simulink model "manometer"  (R2025b)
settings: Solver=VariableStepAuto  StartTime=0.0  StopTime=3600  RelTol=1e-5  AbsTol=1e-7
libraries: fl_lib x17, customization_lib x5, nesl_utility x5
settings Model: Creator=degoede  LastModifiedBy=degoede
settings SolverCC: AutoScaleAbsTol=off
settings SimscapeCC: SimscapeLogType=all  SimscapeLogSimulationStatistics=on  SimscapeLogOpenViewer=on  SimscapeLogLimitData=off

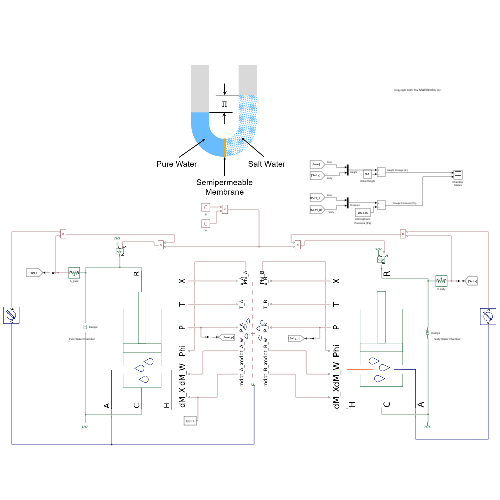
[thumbnail: Simulink's stored preview of the top-level diagram]
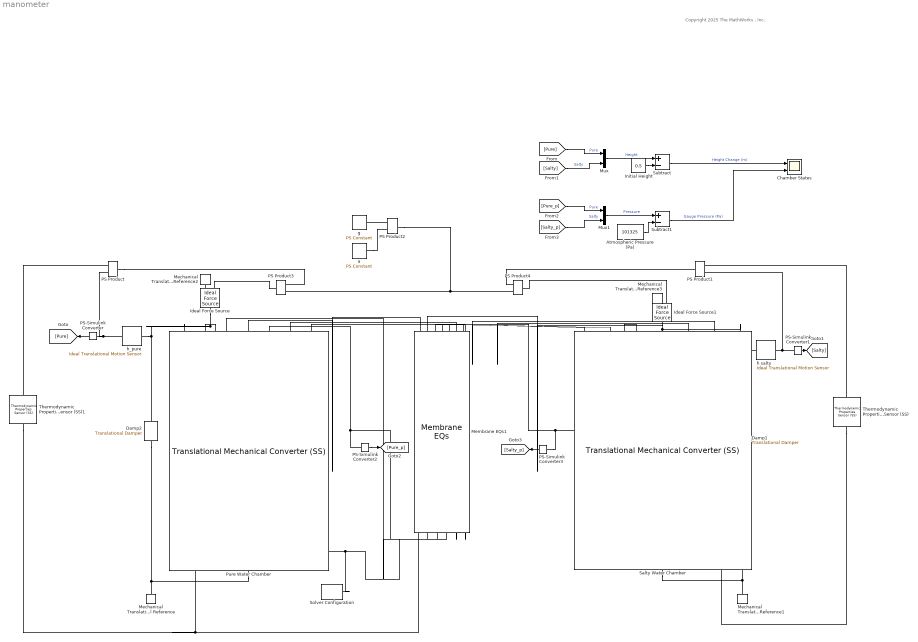
== system manometer ==
  note: Copyright 2025 The MathWorks , Inc.
  Atmospheric Pressure (Pa) : Constant  Value=101325
  Chamber States : Scope  NumInputPorts=2
      settings: Title=Gauge Pressure (Pa)  ActiveDisplayYMinimum=2584.7701229857284  ActiveDisplayYMaximum=6665.5615631627643
  Damp1 : fl_lib/Mechanical/Translational Elements/Translational Damper  D=0.001 N*s/m  v_specify=off  v_priority=None  v=0 m/s  v_nominal_specify=off  v_nominal_value=1  v_nominal_unit=m/s  f_specify=off  f_priority=None  f=0 N  f_nominal_specify=off  f_nominal_value=1  f_nominal_unit=N
  Damp2 : fl_lib/Mechanical/Translational Elements/Translational Damper  D=0.001 N*s/m  v_specify=off  v_priority=None  v=0 m/s  v_nominal_specify=off  v_nominal_value=1  v_nominal_unit=m/s  f_specify=off  f_priority=None  f=0 N  f_nominal_specify=off  f_nominal_value=1  f_nominal_unit=N
  Ideal Force Source : fl_lib/Mechanical/Mechanical Sources/Ideal Force Source
  Ideal Force Source1 : fl_lib/Mechanical/Mechanical Sources/Ideal Force Source
  Initial Height : Constant  Value=0.5
  Mechanical Translational Reference{,1..3} (4 alike) : fl_lib/Mechanical/Translational Elements/Mechanical Translational Reference
  Membrane EQs1 : customization_lib/membranes/Membrane EQs  A_w=2.57e-6 m^3/(N*s)  B_s=2.30e-8 m/s  A_m=1 cm^2
      settings: SourceProductName=Customization  InternalSimscapePortConfiguration="{\"Bottom\":[{\"id\":\"mdot_B_x\",\"label\":\"mdot_B_x\",\"type\":\"output\"},{\"id\":\"mdot_B_w\",\"label\":\"mdot_B_w\",\"type\":\"output\"},{\"id\":\"P_B\",\"label\":\"P_B\",\"type\":\"input\"},{\"id\":\"T_B\",\"label\":\"T_B\",\"type\":\"input\"},{\"id\":\"x_B\",\"label\":\"x_B\",\"type\":\"input\"}],\"Left\":[{\"id\":\"F\",\"label\":\"F\",\"type\":\"customization.solution.solution\"}],\"Right\":[{\"id\":\"Phi_A\",\"label\":\"Phi_A\",\"type\":\"output\"},{\"id\":\"Phi_B\",\"label\":\"Phi_B\",\"type\":\"output\"}],\"Top\":[{\"id\":\"mdot_A_x\",\"label\":\"mdot_A_x\",\"type\":\"output\"},{\"id\":\"mdot_A_w\",\"label\":\"mdot_A_w\",\"type\":\"output\"},{\"id\":\"P_A\",\"label\":\"P_A\",\"type\":\"input\"},{\"id\":\"T_A\",\"label\":\"T_A\",\"type\":\"input\"},{\"id\":\"x_A\",\"label\":\"x_A\",\"type\":\"input\"}]}"
  Mux : Mux  Inputs=2
  Mux1 : Mux  Inputs=2
  PS Product{,1..4} (5 alike) : fl_lib/Physical Signals/Functions/PS Product
  PS-Simulink Converter : nesl_utility/PS-Simulink Converter  PhysicalDomain=network_engine_domain  SubClassName=ps_output  LeftPortType=input  RightPortType=output  PseudoPeriodic=off  Frequencies=[]  VectorFormat=inherit  Unit=m  AffineConversion=off
  PS-Simulink Converter1 : nesl_utility/PS-Simulink Converter  PhysicalDomain=network_engine_domain  SubClassName=ps_output  LeftPortType=input  RightPortType=output  PseudoPeriodic=off  Frequencies=[]  VectorFormat=inherit  Unit=m  AffineConversion=off
  PS-Simulink Converter2 : nesl_utility/PS-Simulink Converter  PhysicalDomain=network_engine_domain  SubClassName=ps_output  LeftPortType=input  RightPortType=output  PseudoPeriodic=off  Frequencies=[]  VectorFormat=inherit  Unit=Pa  AffineConversion=off
  PS-Simulink Converter3 : nesl_utility/PS-Simulink Converter  PhysicalDomain=network_engine_domain  SubClassName=ps_output  LeftPortType=input  RightPortType=output  PseudoPeriodic=off  Frequencies=[]  VectorFormat=inherit  Unit=Pa  AffineConversion=off
  Pure Water Chamber : customization_lib/solution/elements/Translational Mechanical Converter (SS)  mech_orientation=foundation.enum.MechOrientationTranslational.Positive  length_init=0.5 m  interface_area=1 cm^2  dead_volume=1e-07 m^3  area_A=1 cm^2  pressure_spec=foundation.enum.pressure_spec.atmospheric  environment_pressure=0.101325 MPa  m_measure=false  p_measure=true  t_measure=true  x_measure=true  p_I_specify=on  p_I_priority=High  p_I=998.2*9.81*0.5/1e6 + 0.101325 MPa  p_I_nominal_specify=off  p_I_nominal_value=1  p_I_nominal_unit=MPa  T_I_specify=off  T_I_priority=High  T_I=293.15 K  T_I_nominal_specify=off  T_I_nominal_value=1  T_I_nominal_unit=K  x_I_specify=on  x_I_priority=High  x_I=0 kg/m^3  x_I_nominal_specify=off  x_I_nominal_value=1  x_I_nominal_unit=kg/m^3
      settings: SourceProductName=Customization  InternalSimscapePortConfiguration="{\"Bottom\":[{\"id\":\"dM_X\",\"label\":\"dM_X\",\"type\":\"input\"},{\"id\":\"dM_W\",\"label\":\"dM_W\",\"type\":\"input\"},{\"id\":\"Phi\",\"label\":\"Phi\",\"type\":\"input\"},{\"id\":\"P\",\"label\":\"P\",\"type\":\"output\"},{\"id\":\"T\",\"label\":\"T\",\"type\":\"output\"},{\"id\":\"X\",\"label\":\"X\",\"type\":\"output\"}],\"Left\":[{\"id\":\"A\",\"label\":\"A\",\"type\":\"customization.solution.solution\"},{\"id\":\"C\",\"label\":\"C\",\"type\":\"foundation.mechanical.translational.translational\"},{\"id\":\"H\",\"label\":\"H\",\"type\":\"foundation.thermal.thermal\"}],\"Right\":[{\"id\":\"R\",\"label\":\"R\",\"type\":\"foundation.mechanical.translational.translational\"}],\"Top\":[]}"
  Salty Water Chamber : customization_lib/solution/elements/Translational Mechanical Converter (SS)  mech_orientation=foundation.enum.MechOrientationTranslational.Positive  length_init=0.5 m  interface_area=1 cm^2  dead_volume=1e-07 m^3  area_A=1 cm^2  pressure_spec=foundation.enum.pressure_spec.atmospheric  environment_pressure=0.101325 MPa  m_measure=false  p_measure=true  t_measure=true  x_measure=true  p_I_specify=on  p_I_priority=High  p_I=998.25*9.81*0.5/1e6 + 0.101325 MPa  p_I_nominal_specify=off  p_I_nominal_value=1  p_I_nominal_unit=MPa  T_I_specify=off  T_I_priority=High  T_I=293.15 K  T_I_nominal_specify=off  T_I_nominal_value=1  T_I_nominal_unit=K  x_I_specify=on  x_I_priority=High  x_I=0.05 kg/m^3  x_I_nominal_specify=off  x_I_nominal_value=1  x_I_nominal_unit=kg/m^3
      settings: SourceProductName=Customization  InternalSimscapePortConfiguration="{\"Bottom\":[{\"id\":\"dM_X\",\"label\":\"dM_X\",\"type\":\"input\"},{\"id\":\"dM_W\",\"label\":\"dM_W\",\"type\":\"input\"},{\"id\":\"Phi\",\"label\":\"Phi\",\"type\":\"input\"},{\"id\":\"P\",\"label\":\"P\",\"type\":\"output\"},{\"id\":\"T\",\"label\":\"T\",\"type\":\"output\"},{\"id\":\"X\",\"label\":\"X\",\"type\":\"output\"}],\"Left\":[{\"id\":\"A\",\"label\":\"A\",\"type\":\"customization.solution.solution\"},{\"id\":\"C\",\"label\":\"C\",\"type\":\"foundation.mechanical.translational.translational\"},{\"id\":\"H\",\"label\":\"H\",\"type\":\"foundation.thermal.thermal\"}],\"Right\":[{\"id\":\"R\",\"label\":\"R\",\"type\":\"foundation.mechanical.translational.translational\"}],\"Top\":[]}"
  Solver Configuration : nesl_utility/Solver Configuration  PhysicalDomain=network_engine_domain  SubClassName=solver  LeftPortType=input  RightPortType=generic  Tones=[]  Harmonics=[]  SimulateNoise=off  Profile=off  UseLocalSampling=off  EnableSwitchedLinearOptims=on  FrequencyDomain=off  UseCCode=off  RelTol=0.001  AbsTol=0.001  MinStep=1e-09  ToWorkspace=off  RevertToSquareIcSolve=off  NumHomotopyIterations=100  PhasorMode=off  PhasorModeNumHarmonics=1  ConsistencySolver=NEWTON_XTOL_AFTER_FTOL  IndexReductionMethod=DerivativeReplacement  DoDC=off  ResidualTolerance=1e-09  ConsistencyTolSource=GLOBAL  ConsistencyAbsTol=0.001  ConsistencyRelTol=0.001  ConsistencyTolFactor=0.001  UseLocalSolver=off  LocalSolverChoice=NE_BACKWARD_EULER_ADVANCER  ResolveIndetEquations=on  FunctionEvalNumThread=1  LocalSolverSampleTime=0.001  DoFixedCost=off  MaxNonlinIter=3  MaxModeIter=2  ComputeImpulses=off  ImpulseIterations=2  LinearAlgebra=auto  LinearAlgebraNumThread=0  EquationFormulation=NE_TIME_EF  DelaysMemoryBudget=1024  AutomaticFiltering=off  FilteringTimeConstant=0.001  PartitionStorageMethod=AS_NEEDED  PartitionMemoryBudget=1024  PartitionMethod=ROBUST  MultibodyUseLocalSolver=off  MultibodyLocalSolverChoice=ODE1  MultibodyLocalSolverSampleTime=0.001
  Subtract : Sum  Inputs=+-
  Subtract1 : Sum  Inputs=+-
  Thermodynamic Properties Sensor (SS) : customization_lib/solution/sensors/Thermodynamic Properties Sensor (SS)
      settings: SourceProductName=Customization  InternalSimscapePortConfiguration="{\"Bottom\":[],\"Left\":[{\"id\":\"A\",\"label\":\"A\",\"type\":\"customization.solution.solution\"}],\"Right\":[{\"id\":\"RHO\",\"label\":\"ρ\",\"type\":\"output\"}],\"Top\":[]}"
  Thermodynamic Properties Sensor (SS)1 : customization_lib/solution/sensors/Thermodynamic Properties Sensor (SS)
      settings: SourceProductName=Customization  InternalSimscapePortConfiguration="{\"Bottom\":[],\"Left\":[{\"id\":\"A\",\"label\":\"A\",\"type\":\"customization.solution.solution\"}],\"Right\":[{\"id\":\"RHO\",\"label\":\"ρ\",\"type\":\"output\"}],\"Top\":[]}"
  a : fl_lib/Physical Signals/Sources/PS Constant  constant=1 cm^2
  g : fl_lib/Physical Signals/Sources/PS Constant  constant=-9.81 m/s^2
  h salty : fl_lib/Mechanical/Mechanical Sensors/Ideal Translational Motion Sensor  reference=foundation.enum.MeasurementReference.absolute  acceleration_port=false  velocity_port=false  position_port=true  offset=0.5 m
      settings: InternalSimscapePortConfiguration="{\"Bottom\":[],\"Left\":[{\"id\":\"R\",\"label\":\"R\",\"type\":\"foundation.mechanical.translational.translational\"}],\"Right\":[{\"id\":\"P\",\"label\":\"P\",\"type\":\"output\"}],\"Top\":[]}"
  h_pure : fl_lib/Mechanical/Mechanical Sensors/Ideal Translational Motion Sensor  reference=foundation.enum.MeasurementReference.absolute  acceleration_port=false  velocity_port=false  position_port=true  offset=0.5 m
      settings: InternalSimscapePortConfiguration="{\"Bottom\":[],\"Left\":[{\"id\":\"R\",\"label\":\"R\",\"type\":\"foundation.mechanical.translational.translational\"}],\"Right\":[{\"id\":\"P\",\"label\":\"P\",\"type\":\"output\"}],\"Top\":[]}"
  wires:
  PS-Simulink Converter/1 -> [Pure]
  PS-Simulink Converter1/1 -> [Salty]
  PS-Simulink Converter2/1 -> [Pure_p]
  Subtract/1 -> Chamber States/1  "Height Change (m)"
  [Pure] -> Mux/1  "Pure"
  [Salty] -> Mux/2  "Salty"
  PS-Simulink Converter3/1 -> [Salty_p]
  Subtract1/1 -> Chamber States/2  "Gauge Pressure (Pa)"
  [Pure_p] -> Mux1/1  "Pure"
  [Salty_p] -> Mux1/2  "Salty"
  Initial Height/1 -> Subtract/2
  Mux/1 -> Subtract/1  "Height"
  Atmospheric Pressure (Pa)/1 -> Subtract1/2
  Mux1/1 -> Subtract1/1  "Pressure"
  connections:
  Thermodynamic Properties Sensor (SS)1/LConn1 -- Membrane EQs1/LConn1 -- Pure Water Chamber/LConn1
  PS-Simulink Converter2/LConn1 -- Membrane EQs1/LConn4 -- Pure Water Chamber/RConn5
  Mechanical Translational Reference/LConn1 -- Pure Water Chamber/LConn2 -- Damp2/RConn1
  Pure Water Chamber/RConn1 -- Ideal Force Source/LConn1 -- Damp2/LConn1 -- h_pure/LConn1
  Mechanical Translational Reference1/LConn1 -- Damp1/RConn1 -- Salty Water Chamber/LConn2
  PS-Simulink Converter3/LConn1 -- Membrane EQs1/RConn5 -- Salty Water Chamber/RConn5
  Ideal Force Source1/LConn1 -- Damp1/LConn1 -- h salty/LConn1 -- Salty Water Chamber/RConn1
  PS-Simulink Converter1/LConn1 -- PS Product1/LConn2 -- h salty/RConn1
  PS Product/RConn1 -- PS Product3/LConn2
  Mechanical Translational Reference2/LConn1 -- Ideal Force Source/RConn2
  PS Product1/RConn1 -- PS Product4/LConn2
  Mechanical Translational Reference3/LConn1 -- Ideal Force Source1/RConn2
  PS-Simulink Converter/LConn1 -- h_pure/RConn1 -- PS Product/LConn2
  Ideal Force Source/RConn1 -- PS Product3/RConn1
  Thermodynamic Properties Sensor (SS)1/RConn1 -- PS Product/LConn1
  Thermodynamic Properties Sensor (SS)/LConn1 -- Salty Water Chamber/LConn1
  Membrane EQs1/LConn6 -- Pure Water Chamber/RConn7
  Membrane EQs1/LConn5 -- Pure Water Chamber/RConn6
  Membrane EQs1/RConn1 -- Pure Water Chamber/RConn4
  Membrane EQs1/LConn3 -- Pure Water Chamber/RConn3
  Solver Configuration/RConn1 -- Membrane EQs1/LConn2 -- Pure Water Chamber/RConn2
  Membrane EQs1/RConn7 -- Salty Water Chamber/RConn7
  Membrane EQs1/RConn6 -- Salty Water Chamber/RConn6
  Membrane EQs1/RConn2 -- Salty Water Chamber/RConn4
  Membrane EQs1/RConn4 -- Salty Water Chamber/RConn3
  Membrane EQs1/RConn3 -- Salty Water Chamber/RConn2
  Thermodynamic Properties Sensor (SS)/RConn1 -- PS Product1/LConn1
  PS Product2/LConn1 -- g/RConn1
  a/RConn1 -- PS Product2/LConn2
  PS Product2/RConn1 -- PS Product4/LConn1 -- PS Product3/LConn1
  PS Product4/RConn1 -- Ideal Force Source1/RConn1
